simulink model "SimBasOwn"  (R2026b)
settings: Solver=VariableStepAuto  StopTime=inf
undefined symbols (not defined in the file): heartbeatBytes, Payload, SampleTime
libraries: uavmavlinklib x5, simulink x1
settings Model: Creator=cfmm  LastModifiedBy=cfmm

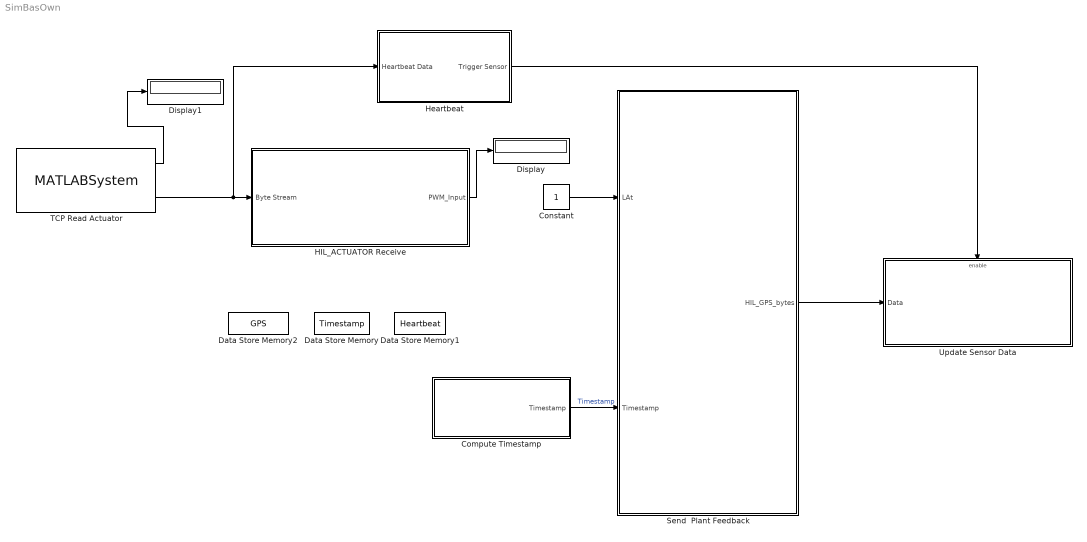
== system SimBasOwn ==
  Compute Timestamp : Subsystem
  Constant : Constant  SampleTime=0.01
  Data Store Memory : DataStoreMemory  DataStoreName=Timestamp  WriteAfterWriteMsg=warning  ShowAdditionalParam=off
  Data Store Memory1 : DataStoreMemory  DataStoreName=Heartbeat  WriteAfterWriteMsg=warning  InitialValue=1  ShowAdditionalParam=off
  Data Store Memory2 : DataStoreMemory  DataStoreName=GPS  WriteAfterWriteMsg=warning  ShowAdditionalParam=off
  Display : Display
  Display1 : Display
  HIL_ACTUATOR Receive : Subsystem
  Heartbeat : Subsystem
  Send  Plant Feedback : Subsystem
  TCP Read Actuator : MATLABSystem  System=px4HostTarget_TCPIP_Read  Length=actuatorBytes  SampleTime=SampleTime
      mask Type: px4HostTarget_TCPIP_Read
  "Update Sensor Data " : Subsystem
  wires:
  Compute Timestamp/1(Timestamp) -> Send  Plant Feedback/2(Timestamp)  "Timestamp"
  TCP Read Actuator/1 -> Display1/1
  HIL_ACTUATOR Receive/1(PWM_Input) -> Display/1
  TCP Read Actuator/2 -> Heartbeat/1(Heartbeat Data), HIL_ACTUATOR Receive/1(Byte Stream)
  Send  Plant Feedback/1(HIL_GPS_bytes) -> "Update Sensor Data "/1(Data)
  Heartbeat/1(Trigger Sensor) -> "Update Sensor Data "/Enable
  Constant/1 -> Send  Plant Feedback/1(LAt)

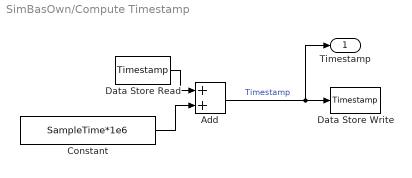
== system SimBasOwn/Compute Timestamp ==
  Add : Sum
  Constant : Constant  Value=SampleTime*1e6  OutDataTypeStr=uint64  SampleTime=SampleTime
  Data Store Read : DataStoreRead  DataStoreName=Timestamp  SampleTime=SampleTime  IndexOptions=Index vector (dialog)  Indices=1  OutputSizes=1
  Data Store Write : DataStoreWrite  DataStoreName=Timestamp  SampleTime=SampleTime  IndexOptions=Index vector (dialog)  Indices=1  OutputSizes=1
  Timestamp : Outport
  wires:
  Data Store Read/1 -> Add/1
  Add/1 -> Timestamp/1, Data Store Write/1  "Timestamp"
  Constant/1 -> Add/2

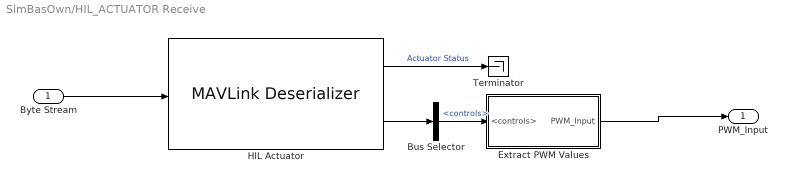
== system SimBasOwn/HIL_ACTUATOR Receive ==
  Byte Stream : Inport
  Bus Selector : BusSelector  OutputSignals=Payload.controls
  Extract PWM Values : Subsystem
  HIL Actuator : uavmavlinklib/MAVLink Deserializer  dialectSource=Specify your own  dialect=common.xml  dialectCustom=/home/cfmm/mypx4/PX4-Autopilot/src/modules/mavlink/mavlink/message_definitions/v1.0/development.xml  version=2  messageType=HIL_ACTUATOR_CONTROLS  inputDataLength=off  SystemIDFilter=off  systemID=1  ComponentIDFilter=off  componentID=1  queueMsg=off  queueMsgSize=50  dropNum=off
  Terminator : Terminator
  PWM_Input : Outport
  wires:
  Byte Stream/1 -> HIL Actuator/1
  HIL Actuator/2 -> Bus Selector/1
  Bus Selector/1 -> Extract PWM Values/1(<controls>)  "<controls>"
  Extract PWM Values/1(PWM_Input) -> PWM_Input/1
  HIL Actuator/1 -> Terminator/1  "Actuator Status"

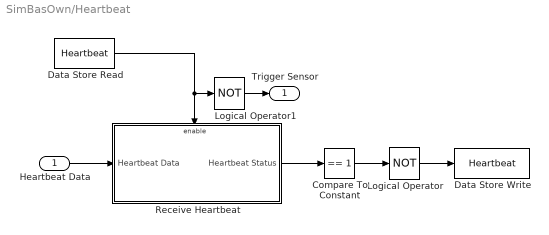
== system SimBasOwn/Heartbeat ==
  Heartbeat Data : Inport
  Compare To Constant : simulink/Logic and Bit Operations/Compare To Constant  relop===  const=1  OutDataTypeStr=uint8
  Data Store Read : DataStoreRead  DataStoreName=Heartbeat  SampleTime=SampleTime  IndexOptions=Index vector (dialog)  Indices=1  OutputSizes=1
  Data Store Write : DataStoreWrite  DataStoreName=Heartbeat  SampleTime=SampleTime  IndexOptions=Index vector (dialog)  Indices=1  OutputSizes=1
  Logical Operator : Logic  Operator=NOT  AllPortsSameDT=off  OutDataTypeStr=boolean
  Logical Operator1 : Logic  Operator=NOT  AllPortsSameDT=off  OutDataTypeStr=boolean
  Receive Heartbeat : Subsystem
  Trigger Sensor : Outport
  wires:
  Logical Operator/1 -> Data Store Write/1
  Data Store Read/1 -> Receive Heartbeat/Enable, Logical Operator1/1
  Receive Heartbeat/1(Heartbeat Status) -> Compare To Constant/1
  Compare To Constant/1 -> Logical Operator/1
  Heartbeat Data/1 -> Receive Heartbeat/1(Heartbeat Data)
  Logical Operator1/1 -> Trigger Sensor/1

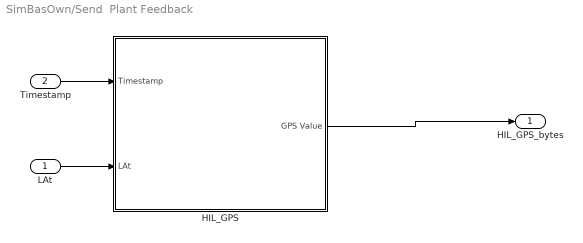
== system SimBasOwn/Send  Plant Feedback ==
  LAt : Inport
  Timestamp : Inport  Port=2
  HIL_GPS : Subsystem
  HIL_GPS_bytes : Outport
  wires:
  Timestamp/1 -> HIL_GPS/1(Timestamp)
  LAt/1 -> HIL_GPS/2(LAt)
  HIL_GPS/1(GPS Value) -> HIL_GPS_bytes/1

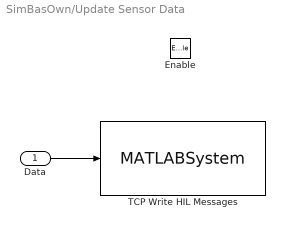
== system SimBasOwn/Update Sensor Data  ==
  Data : Inport
  Enable : EnablePort
  TCP Write HIL Messages : MATLABSystem  System=px4HostTarget_TCPIP_Write
      mask Type: px4HostTarget_TCPIP_Write
  wires:
  Data/1 -> TCP Write HIL Messages/1

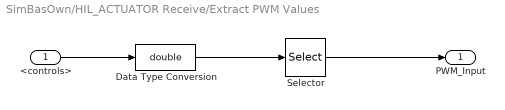
== system SimBasOwn/HIL_ACTUATOR Receive/Extract PWM Values ==
  <controls> : Inport
  Data Type Conversion : DataTypeConversion  OutDataTypeStr=double  SaturateOnIntegerOverflow=off  RndMeth=Floor
  Selector : Selector  InputPortWidth=16  IndexOptions=Index vector (dialog)  Indices=[1:1]  OutputSizes=1  RuntimeRangeChecks=off
  PWM_Input : Outport
  wires:
  Data Type Conversion/1 -> Selector/1
  <controls>/1 -> Data Type Conversion/1
  Selector/1 -> PWM_Input/1

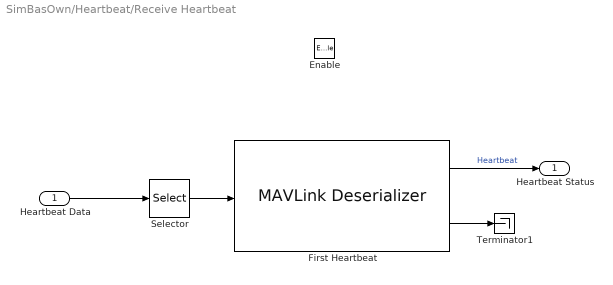
== system SimBasOwn/Heartbeat/Receive Heartbeat ==
  Heartbeat Data : Inport
  Enable : EnablePort
  First Heartbeat : uavmavlinklib/MAVLink Deserializer  dialectSource=Specify your own  dialect=common.xml  dialectCustom=/home/cfmm/mypx4/PX4-Autopilot/src/modules/mavlink/mavlink/message_definitions/v1.0/development.xml  version=2  messageType=HEARTBEAT  inputDataLength=off  SystemIDFilter=off  systemID=1  ComponentIDFilter=off  componentID=1  queueMsg=off  queueMsgSize=50  dropNum=off
  Selector : Selector  InputPortWidth=93  IndexOptions=Index vector (dialog)  Indices=[1:heartbeatBytes]  OutputSizes=1  RuntimeRangeChecks=off
  Terminator1 : Terminator
  Heartbeat Status : Outport
  wires:
  First Heartbeat/2 -> Terminator1/1
  Selector/1 -> First Heartbeat/1
  First Heartbeat/1 -> Heartbeat Status/1  "Heartbeat"
  Heartbeat Data/1 -> Selector/1

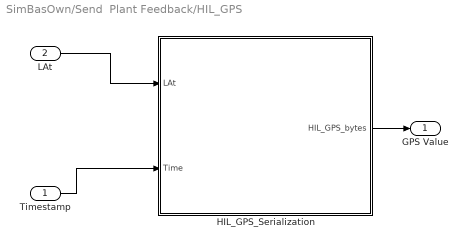
== system SimBasOwn/Send  Plant Feedback/HIL_GPS ==
  Timestamp : Inport
  LAt : Inport  Port=2
  HIL_GPS_Serialization : Subsystem
  GPS Value : Outport
  wires:
  HIL_GPS_Serialization/1(HIL_GPS_bytes) -> GPS Value/1
  LAt/1 -> HIL_GPS_Serialization/1(LAt)
  Timestamp/1 -> HIL_GPS_Serialization/2(Time)

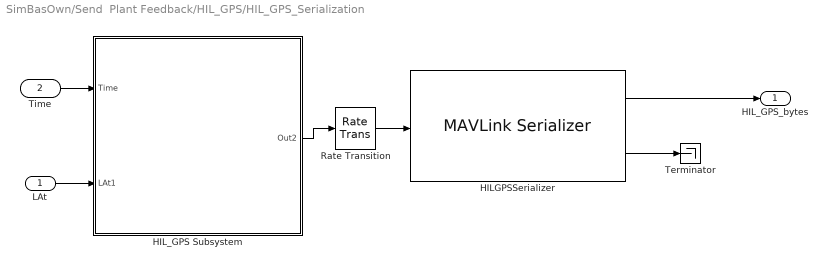
== system SimBasOwn/Send  Plant Feedback/HIL_GPS/HIL_GPS_Serialization ==
  LAt : Inport
  Time : Inport  Port=2
  HILGPSSerializer : uavmavlinklib/MAVLink Serializer  dialectSource=Specify your own  dialect=common.xml  dialectCustom=/home/cfmm/mypx4/PX4-Autopilot/src/modules/mavlink/mavlink/message_definitions/v1.0/development.xml  version=2  messageType=UAM_JOINT_STATES
  HIL_GPS Subsystem : Subsystem
  Rate Transition : RateTransition  OutPortSampleTime=SampleTime
  Terminator : Terminator
  HIL_GPS_bytes : Outport
  wires:
  LAt/1 -> HIL_GPS Subsystem/2(LAt1)
  HILGPSSerializer/2 -> Terminator/1
  HIL_GPS Subsystem/1(Out2) -> Rate Transition/1
  HILGPSSerializer/1 -> HIL_GPS_bytes/1
  Rate Transition/1 -> HILGPSSerializer/1
  Time/1 -> HIL_GPS Subsystem/1(Time)

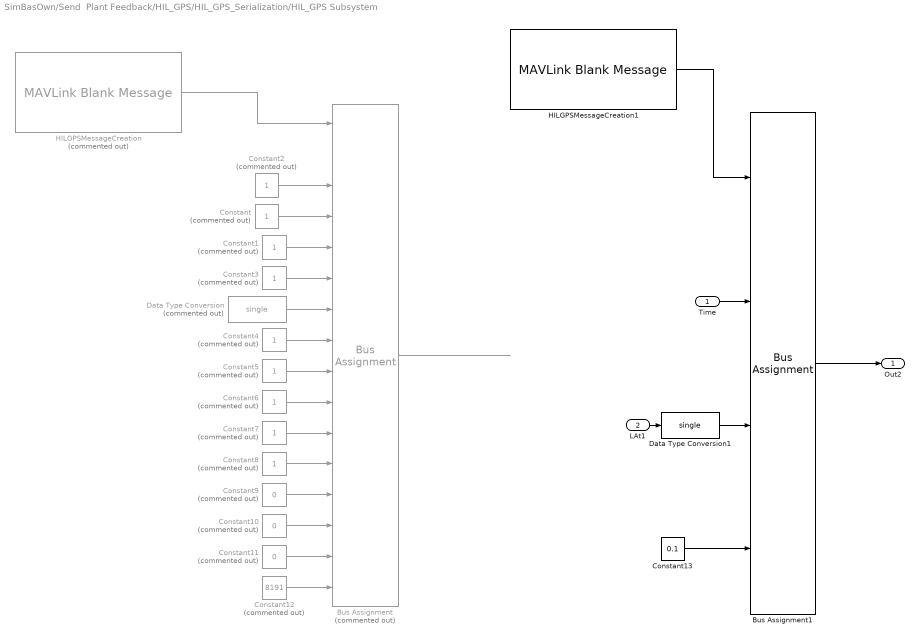
== system SimBasOwn/Send  Plant Feedback/HIL_GPS/HIL_GPS_Serialization/HIL_GPS Subsystem ==
  Time : Inport
  LAt1 : Inport  Port=2
  Bus Assignment : BusAssignment  Commented=on  AssignedSignals=Payload.time_usec,Payload.xacc,Payload.yacc,Payload.zacc,Payload.xgyro,Payload.ygyro,Payload.zgyro,Payload.xmag,Payload.ymag,Payload.zmag,Payload.abs_pressure,Payload.diff_pressure,Payload.pressure_alt,Payload.temperature,Payload.fields_updated
  Bus Assignment1 : BusAssignment  AssignedSignals=Payload.time_usec,Payload.link1_angle,Payload.link2_angle
  Constant{,1..8} (9 alike) : Constant  Commented=on  OutDataTypeStr=single
  Constant10 : Constant  Commented=on  Value=0  OutDataTypeStr=single
  Constant11 : Constant  Commented=on  Value=0  OutDataTypeStr=single
  Constant12 : Constant  Commented=on  Value=8191  OutDataTypeStr=uint32
  Constant13 : Constant  Value=0.1  OutDataTypeStr=single  SampleTime=0.01
  Constant9 : Constant  Commented=on  Value=0  OutDataTypeStr=single
  Data Type Conversion : DataTypeConversion  Commented=on  OutDataTypeStr=single  SaturateOnIntegerOverflow=off  RndMeth=Floor
  Data Type Conversion1 : DataTypeConversion  OutDataTypeStr=single  SaturateOnIntegerOverflow=off  RndMeth=Floor
  HILGPSMessageCreation : uavmavlinklib/MAVLink Blank Message  Commented=on  dialectSource=Select from standard MAVLink dialects  dialect=common.xml  dialectCustom=common.xml  version=2  messageType=HIL_SENSOR  SystemID=2  ComponentID=51  SampleTime=SampleTime
  HILGPSMessageCreation1 : uavmavlinklib/MAVLink Blank Message  dialectSource=Specify your own  dialect=common.xml  dialectCustom=/home/cfmm/mypx4/PX4-Autopilot/src/modules/mavlink/mavlink/message_definitions/v1.0/development.xml  version=2  messageType=UAM_JOINT_STATES  SystemID=2  ComponentID=51  SampleTime=SampleTime
  Out2 : Outport
  wires:
  HILGPSMessageCreation/1 -> Bus Assignment/1
  Bus Assignment/1 -> ?
  Time/1 -> Bus Assignment1/2
  Constant/1 -> Bus Assignment/4
  Constant12/1 -> Bus Assignment/16
  Constant1/1 -> Bus Assignment/5
  Constant2/1 -> Bus Assignment/3
  Constant3/1 -> Bus Assignment/6
  Constant4/1 -> Bus Assignment/8
  Constant5/1 -> Bus Assignment/9
  Constant6/1 -> Bus Assignment/10
  Constant7/1 -> Bus Assignment/11
  Constant8/1 -> Bus Assignment/12
  Constant9/1 -> Bus Assignment/13
  Constant10/1 -> Bus Assignment/14
  Constant11/1 -> Bus Assignment/15
  Data Type Conversion/1 -> Bus Assignment/7
  HILGPSMessageCreation1/1 -> Bus Assignment1/1
  Bus Assignment1/1 -> Out2/1
  LAt1/1 -> Data Type Conversion1/1
  Data Type Conversion1/1 -> Bus Assignment1/3
  Constant13/1 -> Bus Assignment1/4
